simulink model "tractor_mu1109"  (R2022b)
settings: Solver=FixedStepDiscrete  StartTime=0.0  StopTime=20  FixedStep=0.001  RelTol=1e-3
model workspace (MAT data in the model file):
  P : object (value not decoded)
  w_2 : Simulink.Parameter (value not decoded)
undefined symbols (not defined in the file): A, a, B, b, C, D, DiscIntNeverNeededParam, Iz, K, k1, K1, k2, K2, L1, L2, m, magnitude, Phi, Sample_time, Steer_Ratio
libraries: simulink x26, slpidlib x13, Solver_SF x1, dsparch4 x1
(part 5 of 7)

== matlab function tractor_mu1109/Dugoff轮胎模型/pac2002/fr_dugoff ==
  data: Fz input; Fx0 output; u input; lamda input; alpha input; Fy0 output; Fx output; Fy output
function [Fx0,Fy0,Fx,Fy] = tire(Fz,u,lamda,alpha)
cx = -20;
cy = -20;
L = (1-lamda)/(2*sqrt((cx^2)*(lamda^2)+(cy^2)*((tan(alpha))^2)));
if L<1
    fL = L*(2-L);
else
    fL = 1;
end
Fx0 = Fz*cx*lamda*fL/(1-lamda);
Fy0 = Fz*cy*tan(alpha)*fL/(1-lamda);
Fx = u*Fx0;
Fy = u*Fy0;

== matlab function tractor_mu1109/软土分配策略/MATLAB Function1 ==
  data: measured_kappa input; torque_l1_n_m output; baseline_torques_n_m input; wheel_torque_limits_n_m input; torque_r1_n_m output; torque_l2_n_m output; torque_r2_n_m output
function [torque_l1_n_m, torque_r1_n_m, torque_l2_n_m, torque_r2_n_m] = shiche_soft_soil_adaptive_allocation(measured_kappa, baseline_torques_n_m, wheel_torque_limits_n_m)
%SHICHE_SOFT_SOIL_ADAPTIVE_ALLOCATION Direct-slip zero-sum torque allocator.
%
% MATLAB Function block version for real-vehicle VCU code generation. All
% calculations and outputs use single precision.
%
% Wheel vector order:
%   [L1, R1, L2, R2] = [left-front, right-front, left-rear, right-rear]
%
% Inputs:
%   measured_kappa       Directly measured four-wheel longitudinal slip ratios.
%   baseline_torques_n_m Upstream baseline wheel torques in N*m.
%   wheel_torque_limits_n_m Nonnegative maximum wheel torques in N*m.
%
% Outputs:
%   torque_l1_n_m Redistributed left-front wheel torque in N*m.
%   torque_r1_n_m Redistributed right-front wheel torque in N*m.
%   torque_l2_n_m Redistributed left-rear wheel torque in N*m.
%   torque_r2_n_m Redistributed right-rear wheel torque in N*m.
%
% Allocation principle:
%   1. Compare each wheel slip with the four-wheel mean slip.
%   2. Remove torque from wheels with above-average slip and add torque to
%      wheels with below-average slip.
%   3. Limit each wheel's redistribution correction to +/-2600 N*m.
%   4. Force the four correction values to sum to zero, so the final total
%      torque equals the baseline total torque.
%   5. Uniformly reduce the zero-sum correction when needed so every final
%      wheel torque remains between zero and its input wheel torque limit.
%
% This function intentionally contains no slip estimation, adaptive target,
% CBF, QP, or persistent cross-step state.
%
% The baseline allocation is expected to satisfy the input wheel limits. If
% the baseline itself is outside those limits, preserving its total torque and
% satisfying every wheel limit may be impossible. In that case this function
% returns the baseline unchanged and performs no slip redistribution.

slips = reshape(single(measured_kappa), 1, 4);
base_torques = reshape(single(baseline_torques_n_m), 1, 4);
wheel_limits = reshape(single(wheel_torque_limits_n_m), 1, 4);

feedback_gain_n_m = single(20500.0);
correction_limit_n_m = single(2600.0);
corrections = zeros(1, 4, 'single');

% Invalid direct-slip or limit input must not corrupt the baseline allocation.
inputs_valid = true;
baseline_within_limits = true;
for index = 1:4
    if ~isfinite(slips(index)) || ~isfinite(wheel_limits(index)) ...
            || wheel_limits(index) < single(0.0)
        inputs_valid = false;
    end
    if ~isfinite(base_torques(index)) || base_torques(index) < single(0.0) ...
            || base_torques(index) > wheel_limits(index)
        baseline_within_limits = false;
    end
end

if inputs_valid && baseline_within_limits
    mean_slip = sum(slips) / single(4.0);

    % Initial proportional redistribution. Positive slip deviation removes
    % torque; negative slip deviation adds torque.
    for index = 1:4
        slip_deviation = slips(index) - mean_slip;
        corrections(index) = clamp_local( ...
            -feedback_gain_n_m * slip_deviation, ...
            -correction_limit_n_m, ...
            correction_limit_n_m);
    end

    % Independent saturation can make the corrections non-zero-sum. Center
    % them again so torque removed from high-slip wheels is exactly reassigned
    % to lower-slip wheels.
    mean_correction = sum(corrections) / single(4.0);
    for index = 1:4
        corrections(index) = corrections(index) - mean_correction;
    end

    % Re-centering can increase one correction beyond the requested limit.
    % Uniform scaling preserves the zero-sum property and relative allocation.
    maximum_abs_correction = single(0.0);
    for index = 1:4
        maximum_abs_correction = max( ...
            maximum_abs_correction, abs(corrections(index)));
    end
    if maximum_abs_correction > correction_limit_n_m
        scale = correction_limit_n_m / maximum_abs_correction;
        corrections = corrections * scale;
    end

    % Apply one common scale to all corrections so the zero-sum transfer and
    % total baseline torque are preserved while respecting every wheel limit.
    bound_scale = single(1.0);
    for index = 1:4
        if corrections(index) > single(0.0)
            available_increase = wheel_limits(index) - base_torques(index);
            bound_scale = min(bound_scale, available_increase / corrections(index));
        elseif corrections(index) < single(0.0)
            available_decrease = base_torques(index);
            bound_scale = min(bound_scale, available_decrease / -corrections(index));
        end
    end
    bound_scale = clamp_local(bound_scale, single(0.0), single(1.0));
    corrections = corrections * bound_scale;
end

selected_torques = base_torques + corrections;

% Compensate the small single-precision summation residual on a wheel that has
% room in the required direction, without violating an input torque limit.
total_residual = sum(base_torques) - sum(selected_torques);
if inputs_valid && baseline_within_limits && total_residual ~= single(0.0)
    for index = 1:4
        corrected = selected_torques(index) + total_residual;
        if corrected >= single(0.0) && corrected <= wheel_limits(index)
            selected_torques(index) = corrected;
            break;
        end
    end
end

torque_l1_n_m = single(selected_torques(1));
torque_r1_n_m = single(selected_torques(2));
torque_l2_n_m = single(selected_torques(3));
torque_r2_n_m = single(selected_torques(4));
end

function value = clamp_local(value_in, lower, upper)
value = min(max(single(value_in), single(lower)), single(upper));
end

== matlab function tractor_mu1109/软土扭矩分配/状态接口与轮端动力学 ==
  data: wheel_speeds_rpm input; kappa output; front_steer_angles_deg input; longitudinal_speed_mps input; slip_ratios input; slip_ratio_dots input; slip_valid input; baseline_torques_n_m input; wheel_torque_limits_n_m input; dot_kappa output; kappa_valid output; wheel_omegas_radps output; rolling_speeds_mps output; surface_speeds_mps output; front_steers_rad output; base_torques_n_m output; wheel_limits_n_m output; input_gains output
function [kappa, dot_kappa, kappa_valid, wheel_omegas_radps, rolling_speeds_mps, surface_speeds_mps, front_steers_rad, base_torques_n_m, wheel_limits_n_m, input_gains] = MF_StateKinematicsAndGain(wheel_speeds_rpm, front_steer_angles_deg, longitudinal_speed_mps, slip_ratios, slip_ratio_dots, slip_valid, baseline_torques_n_m, wheel_torque_limits_n_m)

% 状态接口与轮端运动学模块
%
% 本模块不再内部估计滑移率。
% 滑移率、滑移率变化率以及滑移率有效标志均由外部状态估计模块输入。
%
% 四轮顺序：
% 1：左前轮
% 2：右前轮
% 3：左后轮
% 4：右后轮

%% 输入整理

wheel_speeds = row4_local(wheel_speeds_rpm);
kappa_input = row4_local(slip_ratios);
dot_kappa_input = row4_local(slip_ratio_dots);
valid_input = row4_local(slip_valid);
base_input = row4_local(baseline_torques_n_m);
limit_input = row4_local(wheel_torque_limits_n_m);

vx = double(longitudinal_speed_mps);

%% 前轮转角整理

front_steers_rad = front_steer_pair_rad_local(front_steer_angles_deg);

%% 基本车辆参数

rpm_to_rad = 2.0 * pi / 60.0;

radii = [0.834, 0.834, 0.94, 0.94];
inertias = [110.64, 110.64, 356.42, 356.42]; % 转动惯量

%% 滑移率外部输入整理

kappa = zeros(1, 4);
dot_kappa = zeros(1, 4);
kappa_valid = zeros(1, 4);

for index = 1:4

    % 外部滑移率直接使用，但做基本数值限幅，防止异常值进入控制器。
    kappa(index) = clamp_local(kappa_input(index), -1.0, 1.0);

    % 外部滑移率变化率直接使用。
    dot_kappa(index) = dot_kappa_input(index);

    % 有效性由外部 slip_valid 给出，同时内部补充有限性检查。
    if valid_input(index) > 0.5 && isfinite(kappa(index)) && isfinite(dot_kappa(index))
        kappa_valid(index) = 1.0;
    else
        kappa_valid(index) = 0.0;
        dot_kappa(index) = 0.0;
    end
end

%% 轮端运动学计算

% 轮速由 rpm 转为 rad/s。
wheel_omegas_radps = abs(wheel_speeds) * rpm_to_rad;

% 车轮圆周速度 v = r * omega。
surface_speeds_mps = radii .* wheel_omegas_radps;

% 车速取绝对值，避免倒车时符号影响滑移率输入增益计算。
speed_abs = abs(vx);

% 前轮转角。
delta_l = front_steers_rad(1);
delta_r = front_steers_rad(2);

% 各轮沿滚动方向的车辆速度。
% 前轮考虑转角投影，后轮无转角。
rolling_speeds_mps = zeros(1, 4);
rolling_speeds_mps(1) = abs(speed_abs * cos(delta_l));
rolling_speeds_mps(2) = abs(speed_abs * cos(delta_r));
rolling_speeds_mps(3) = speed_abs;
rolling_speeds_mps(4) = speed_abs;

%% 基线扭矩与轮端限幅整理

wheel_limits_n_m = zeros(1, 4);
base_torques_n_m = zeros(1, 4);

for index = 1:4

    % 轮端最大扭矩不能为负。
    wheel_limits_n_m(index) = max(0.0, limit_input(index));

    % 基线扭矩限制在物理可行范围内。
    base_torques_n_m(index) = clamp_local(base_input(index), 0.0, wheel_limits_n_m(index));
end

%% 滑移率动力学输入增益计算

% 滑移率动力学近似写为：
% dot(kappa_i) = g_i * T_i + d_i
%
% 其中：
% g_i = v_i / (J_i * r_i * omega_i^2)

input_gains = NaN(1, 4);

for index = 1:4

    if kappa_valid(index) > 0.5 && wheel_omegas_radps(index) > 0.0 && isfinite(rolling_speeds_mps(index))

        gain = rolling_speeds_mps(index) / ...
            (inertias(index) * radii(index) * wheel_omegas_radps(index) * wheel_omegas_radps(index));

        if gain >= 1.0e-8 && isfinite(gain)
            input_gains(index) = gain;
        end
    end
end

end


function output = row4_local(values)

% 将输入信号整理为 1×4 行向量。

input_values = double(values);
output = zeros(1, 4);

for index = 1:4
    output(index) = input_values(index);
end

end


function front_steers_rad = front_steer_pair_rad_local(front_steer_angles_deg)

% 将前轮转角输入整理为左右前轮两个转角，单位 rad。
% 如果输入为两个元素，则分别为左前轮和右前轮转角；
% 如果输入为一个元素，则左右前轮使用同一等效转角。

steer_input = double(front_steer_angles_deg);
front_steers_rad = zeros(1, 2);

if numel(steer_input) >= 2
    front_steers_rad(1) = steer_input(1) * pi / 180.0;
    front_steers_rad(2) = steer_input(2) * pi / 180.0;
else
    front_steers_rad(1) = steer_input(1) * pi / 180.0;
    front_steers_rad(2) = steer_input(1) * pi / 180.0;
end

end


function value = clamp_local(value_in, lower, upper)

% 数值限幅函数。

value = min(max(double(value_in), double(lower)), double(upper));

end

== matlab function tractor_mu1109/四轮转矩分配/基线垂直载荷分配 ==
  data: Mz input; Tfl output; Tfr output; Trl output; Trr output; T0 input; derta input; k input; mode input
function [Tfl,Tfr,Trl,Trr] = fcn(Mz,T0,derta,k,mode)
rf = single(0.834);
rr = single(0.94);
df = single(2.39);
dr = single(2.33);
a = single(2.043);

Trr = single(0);
Trl = single(0);
Tfl = single(0);
Tfr = single(0);


% 强制将输入 Mz 类型设为 single，避免隐式转换
Mz = single(Mz);
T0 = single(T0);
derta = single(derta);
mode = single(mode);

% if mode == 5 || mode == 6
%     k = single(3/7); 
% elseif mode == 1 || mode == 3 
%     k = min(k,1);
%     k = max(k,0.3);
% end

A = T0 / (k + single(1));
B = (Mz - a*sin(derta)*k*A/rf) / (df*cos(derta)*k*rr + dr*rf) * (2*rf*rr);
Trr = (A + B) / single(2);
Trl = (A - B) / single(2);
Tfl = k * Trl;
Tfr = k * Trr;

== matlab function tractor_mu1109/牵引效率计算/右后轮 ==
  data: Tw input; Fx_est output; omega_meas input; Fz input; Fx_raw output; Fx_limited output; omega_hat_out output; e_omega output; wv output
function [Fx_est, Fx_raw, Fx_limited, omega_hat_out, e_omega, wv] = ...
    RearWheelFxObserver(Tw, omega_meas, Fz)

%#codegen
% 单轮纵向驱动力观测器
% 输入仅保留时变信号：
%   Tw         : 轮端驱动力矩 [N*m]
%   omega_meas : 实测车轮角速度 [rad/s]
%   Fz         : 单轮垂直载荷 [N]
%
% 输出：
%   Fx_est        : 最终纵向驱动力估计 [N]
%   Fx_raw        : 原始观测力估计 [N]
%   Fx_limited    : 限幅后力估计 [N]
%   omega_hat_out : 观测器内部估计轮速 [rad/s]
%   e_omega       : 轮速误差 [rad/s]
%   wv            : 低速平滑权重 [-]

% =========================================================
% 1. 固定参数区：根据具体车轮统一在这里调整
% =========================================================

Re = 0.94;              % 有效滚动半径 [m]
Jw = 356.42;            % 车轮等效转动惯量 [kg*m^2]
Ts = 0.001;             % 采样周期 [s]

mu = 0.7;               % 等效附着系数 [-]

l_omega = 50.0;         % 轮速误差反馈增益
fF = 3.0;               % 轮胎力观测带宽 [Hz]
gamma_F = Jw / Re * (2*pi*fF)^2;

enable_smc = 0;         % 是否启用滑模鲁棒项：1启用，0关闭
phi = 1.5;              % 滑模边界层厚度 [rad/s]
Func_ratio = 0.10;      % 未建模力比例，建议0.05~0.20
ks = Re / Jw * Func_ratio * mu * max(Fz, 0.0);

enable_lpf = 0;         % 是否启用输出低通：1启用，0关闭
tau_F = 0.08;           % 输出低通时间常数 [s]

v0 = 0.10;              % 低速权重起点 [m/s]
v1 = 0.80;              % 低速权重终点 [m/s]

eps_neg = 0.0;          % 允许负驱动力比例；严格驱动力估计取0
T_offset = 0.0;         % 轮端扭矩零偏 [N*m]
T_dead = 10.0;          % 扭矩死区 [N*m]

allow_brake_force = 0;  % 0：只估计驱动力；1：允许估计制动力

% =========================================================
% 2. 持久状态变量
% =========================================================

persistent omega_hat
persistent Fx_hat
persistent Fx_filt
persistent initialized

if isempty(initialized)
    omega_hat = 0.0;
    Fx_hat = 0.0;
    Fx_filt = 0.0;
    initialized = false;
end

if ~initialized
    omega_hat = omega_meas;
    Fx_hat = 0.0;
    Fx_filt = 0.0;
    initialized = true;
end

% =========================================================
% 3. 参数保护
% =========================================================

Jw_safe = max(Jw, 1e-6);
Re_safe = max(Re, 1e-6);
Ts_safe = max(Ts, 1e-6);
phi_safe = max(phi, 1e-6);
tau_safe = max(tau_F, Ts_safe);

Fz_safe = max(Fz, 0.0);
mu_safe = max(mu, 0.0);

if v1 <= v0
    v1_safe = v0 + 1e-3;
else
    v1_safe = v1;
end

% =========================================================
% 4. 扭矩零偏与死区处理
% =========================================================

Tw_corr = Tw - T_offset;

if abs(Tw_corr) < T_dead
    Tw_eff = 0.0;
else
    if Tw_corr > 0.0
        Tw_eff = Tw_corr - T_dead;
    else
        Tw_eff = Tw_corr + T_dead;
    end
end

if allow_brake_force < 0.5
    if Tw_eff < 0.0
        Tw_eff = 0.0;
    end
end

% =========================================================
% 5. 轮速误差
% =========================================================

e_omega = omega_meas - omega_hat;

% =========================================================
% 6. 滑模鲁棒项
% =========================================================

s = e_omega / phi_safe;

if s > 1.0
    sat_s = 1.0;
elseif s < -1.0
    sat_s = -1.0;
else
    sat_s = s;
end

if enable_smc > 0.5
    smc_term = ks * sat_s;
else
    smc_term = 0.0;
end

% =========================================================
% 7. 观测器状态更新
% =========================================================
%
% omega_hat_dot = Tw/Jw - Re/Jw*Fx_hat + l_omega*e_omega + ks*sat(e/phi)
% Fx_hat_dot    = -gamma_F*e_omega

omega_hat_dot = ...
    Tw_eff / Jw_safe ...
    - Re_safe / Jw_safe * Fx_hat ...
    + l_omega * e_omega ...
    + smc_term;

Fx_hat_dot = -gamma_F * e_omega;

omega_hat = omega_hat + Ts_safe * omega_hat_dot;
Fx_hat = Fx_hat + Ts_safe * Fx_hat_dot;

% =========================================================
% 8. 物理限幅与抗积分发散
% =========================================================

Fx_max = mu_safe * Fz_safe;

if allow_brake_force > 0.5
    Fx_min = -mu_safe * Fz_safe;
else
    Fx_min = -eps_neg * Fz_safe;
end

if Fx_hat > Fx_max
    Fx_hat = Fx_max;
elseif Fx_hat < Fx_min
    Fx_hat = Fx_min;
end

Fx_raw = Fx_hat;

if Fx_raw > Fx_max
    Fx_limited = Fx_max;
elseif Fx_raw < Fx_min
    Fx_limited = Fx_min;
else
    Fx_limited = Fx_raw;
end

% =========================================================
% 9. 低速平滑权重
% =========================================================

vw = abs(Re_safe * omega_meas);

wv = (vw - v0) / (v1_safe - v0);

if wv > 1.0
    wv = 1.0;
elseif wv < 0.0
    wv = 0.0;
end

wv = wv * wv * (3.0 - 2.0 * wv);

Fx_weighted = wv * Fx_limited;

% =========================================================
% 10. 输出低通滤波
% =========================================================

if enable_lpf > 0.5
    alpha = exp(-Ts_safe / tau_safe);
    Fx_filt = alpha * Fx_filt + (1.0 - alpha) * Fx_weighted;
    Fx_est = Fx_filt;
else
    Fx_filt = Fx_weighted;
    Fx_est = Fx_weighted;
end

omega_hat_out = omega_hat;

end

== matlab function tractor_mu1109/Dugoff轮胎模型/pac2002/rl_dugoff ==
  data: Fz input; Fx0 output; u input; lamda input; alpha input; Fy0 output; Fx output; Fy output
function [Fx0,Fy0,Fx,Fy] = tire(Fz,u,lamda,alpha)
cx = -20;
cy = -20;
L = (1-lamda)/(2*sqrt(cx^2*lamda^2+cy^2*(tan(alpha))^2));
if L<1
    fL = L*(2-L);
else
    fL = 1;
end
Fx0 = Fz*cx*lamda*fL/(1-lamda);
Fy0 = Fz*cy*tan(alpha)*fL/(1-lamda);
Fx = u*Fx0;
Fy = u*Fy0;

== matlab function tractor_mu1109/Dugoff轮胎模型/pac2002/rr_dugoff ==
  data: Fz input; Fx0 output; u input; lamda input; alpha input; Fy0 output; Fx output; Fy output
function [Fx0,Fy0,Fx,Fy] = tire(Fz,u,lamda,alpha)
cx = -20;
cy = -20;
L = (1-lamda)/(2*sqrt((cx^2)*(lamda^2)+(cy^2)*((tan(alpha))^2)));
if L<1
    fL = L*(2-L);
else
    fL = 1;
end
Fx0 = Fz*cx*lamda*fL/(1-lamda);
Fy0 = Fz*cy*tan(alpha)*fL/(1-lamda);
Fx = u*Fx0;
Fy = u*Fy0;

== matlab function tractor_mu1109/质心侧偏角估计/define_Kalman ==
  data: u input; A output; B output; C output; D output; a11 output; a12 output; a21 output single; a22 output; c11 output; c12 output
function [A, B, C, D,a11,a12,a21,a22,c11,c12] = fcn(u)
m = 18530;%质量
Iz = 67536;%绕Z轴的转动惯量
a = 2.043;%前轴距
b=1.362;%后轴距
% k1 = -1360400;%前侧偏刚度
% k2 = -1611200;%后侧偏刚度
k1 = -304828*2;%前侧偏刚度
k2 = -417040*2;%后侧偏刚度
t = 0.001;%仿真步长
Sample_time = 0.001;


a11 = (k1+k2)*t/(m*u)+1;
a12 = ((a*k1-b*k2)/(m*u^2)-1)*t;
a21 = single((a*k1-b*k2)*t/Iz);
a22 = (a^2*k1+b^2*k2)*t/(Iz*u)+1;
b11  =-k1*t/(m*u);
b21 = -a*k1*t/Iz;
c11 = (k1+k2)/m;
c12 = (a*k1-b*k2)/(m*u);
c21 = 0;
c22 = 1;
d11 = -k1/m;
d21 = 0;

%% A B C D 为kalman滤波器中各个矩阵

A = [a11 a12;a21 a22];
B = [b11;b21];
C = [c11 c12;c21 c22];
D = [d11;d21];

== matlab function tractor_mu1109/驱动防滑模块/MATLAB Function ==
  data: sp1 input; vfl output; sp2 input; vfr output
function [vfl,vfr] = fcn(sp1,sp2)
r1 = 0.834;

if sp1>=0
    vfl = max(0.001,sp1*2*pi*r1/60); %m/s
else
    vfl = min(-0.001,sp1*2*pi*r1/60); %m/s
end

if sp2 >= 0
    vfr = max(0.001,sp2*2*pi*r1/60);
else
    vfr = min(0.001,sp2*2*pi*r1/60);
end

== matlab function tractor_mu1109/驱动防滑模块/MATLAB Function1 ==
  data: sp3 input; vrl output; sp4 input; vrr output
function [vrl,vrr] = fcn(sp3,sp4)
r2 = 0.94;

if sp3 >= 0
    vrl = max(0.001,sp3*2*pi*r2/60);
else
    vrl = min(0.001,sp3*2*pi*r2/60);
end

if sp4 >=0
    vrr = max(0.001,sp4*2*pi*r2/60);
else
    vrr = min(0.001,sp4*2*pi*r2/60);
end

== stateflow chart tractor_mu1109/驱动防滑模块/转矩协调控制 ==
  state coordinate
    (default) -> (junction 7)
    (junction 7) -> (junction 9) [order 1] : [dT1 ~= 0]
    (junction 9) -> (junction 11) [order 1] : [dT2 ~= 0]
    (junction 11) -> (junction 14) [order 1] : [abs(dT1)>=abs(dT2)]{dTfr=dT1;dTfl=dT1;}
    (junction 14) -> (junction 16)
    (junction 7) -> (junction 21) [order 2] : {dTfr=dT2;
        | dTfl=dT2}
    (junction 9) -> (junction 19) [order 2] : {dTfr=dT1;
        | dTfl=dT1;}
    (junction 11) -> (junction 16) [order 2] : {dTfr=dT2;dTfl=dT2;}
    (junction 19) -> (junction 21)
    (junction 16) -> (junction 19)
    (junction 21) -> (junction 111)
    (junction 111) -> (junction 106) [order 2] : {dTrr=dT4;
        | dTrl=dT4}
    (junction 111) -> (junction 118) [order 1] : [dT3 ~= 0]
    (junction 118) -> (junction 107) [order 1] : [dT4 ~= 0]
    (junction 107) -> (junction 110) [order 1] : [abs(dT3)>=abs(dT4)]{dTrr=dT3;dTrl=dT3;}
    (junction 110) -> (junction 114)
    (junction 115) -> (junction 106)
    (junction 118) -> (junction 115) [order 2] : {dTrr=dT3;
        | dTrl=dT3;}
    (junction 107) -> (junction 114) [order 2] : {dTrr=dT4;dTrl=dT4;}
    (junction 114) -> (junction 115)
  state no_coordinate
    du:
    dTfl=dT1;
    dTfr=dT2;
    dTrl=dT3;
    dTrr=dT4;
  (default) -> (junction 123)
  (junction 123) -> (junction 126) [order 2]
  (junction 123) -> no_coordinate [order 1] : [v<10]
  (junction 126) -> coordinate
  no_coordinate -> coordinate : [v>=10]
  coordinate -> no_coordinate [order 1] : [v<10]
  coordinate -> coordinate [order 2] : [v>=10]
  data: v input; dT1 input; dT2 input; dT3 input; dT4 input; dTfl output; dTfr output; dTrl output; dTrr output

== matlab function tractor_mu1109/四轮转矩分配/MATLAB Function1 ==
  data: X_current input; U_optimal output; Fx input; Mz input; Fz_all input; mu input; last_U_in input
function U_optimal = mpc_torque_allocation_fcn(X_current, Fx, Mz, Fz_all, mu, last_U_in)
% 基于MPC的四轮驱动车辆扭矩分配。
% 本函数在每个计算步中构建并求解一个二次规划(QP)问题。

%#codegen

% -------------------------------------------------------------------------
% 1. 定义持久化变量和参数
% -------------------------------------------------------------------------
% persistent 关键字定义的变量只在第一次调用函数时初始化，之后会保持它们的值。
persistent vehicle_params mpc_params last_U

if isempty(vehicle_params)
    % --- 车辆参数 ---
    % !! 请根据您的拖拉机模型修改以下参数 !!
    vehicle_params.m = 18530;   % 质量 (kg)
    vehicle_params.Iz = 67536;  % 绕Z轴的转动惯量 (kg*m^2)
    vehicle_params.lf = 2.043;   % 质心到前轴的距离 (m)
    vehicle_params.lr = 1.362;   % 质心到后轴的距离 (m)
    vehicle_params.wf = 2.39;    % 前轮距 (m)
    vehicle_params.wr = 2.33;    % 后轮距 (m)

    % --- MPC 参数 ---
    mpc_params.Ts = 0.001;      % 采样时间 (s)，必须与Simulink的采样时间一致
    mpc_params.Np = 20;        % 预测时域 (Prediction Horizon)
    mpc_params.Nc = 10;         % 控制时域 (Control Horizon)
    
    % --- MPC 权重 ---
    % 对控制输入变化率 (delta U) 的惩罚矩阵R的对角线元素
    mpc_params.R_diag = ones(8, 1) * 0.01; 
    mpc_params.w_ax = 1.0;      % 纵向加速度权重
    mpc_params.w_ay = 1;      % 横向加速度权重
    
    % --- 轮胎附着多边形 ---
    % 使用一个八边形来线性化近似摩擦圆约束
    num_sides = 8;
    angles = (0:num_sides-1)' * (2*pi/num_sides);
    mpc_params.friction_polygon = [cos(angles), sin(angles)]; % [cos, sin] 列
    
    % 初始化上一次的控制输入
    last_U = zeros(8, 1);
end

% 从输入端口更新last_U，以保证时间步之间的一致性
if any(size(last_U_in) ~= size(last_U))
   last_U = zeros(8,1); % 如果是第一次运行或尺寸不匹配，则进行初始化
else
   last_U = last_U_in;
end


% -------------------------------------------------------------------------
% 2. 获取参数
% -------------------------------------------------------------------------
% 车辆参数
m = vehicle_params.m;
Iz = vehicle_params.Iz;
lf = vehicle_params.lf;
lr = vehicle_params.lr;
wf = vehicle_params.wf;
wr = vehicle_params.wr;
bf = wf / 2; % 半轮距
br = wr / 2;

% MPC参数
Ts = mpc_params.Ts;
Np = mpc_params.Np;
Nc = mpc_params.Nc;
R = diag(mpc_params.R_diag);

% 解析输入信号
u_k = X_current(1); % 当前的纵向车速 (m/s)
v_k = X_current(2); % 当前的横向车速 (m/s)
r_k = X_current(3); % 当前横摆角速度 (rad/s)

% -------------------------------------------------------------------------
% 3. 定义状态空间矩阵 
% -------------------------------------------------------------------------
% 连续时间的状态矩阵 A_c，它依赖于当前车速 u_k
A_c = [0, 0, 0;
       0, 0, u_k;
       0, 0, 0];

% 连续时间的输入矩阵 B_c  横摆方向逆时针为正;横向向左为正
B_c = [1/m,   0,   1/m,   0,   1/m,   0,   1/m,   0;
       0,   1/m,   0,   1/m,   0,   1/m,   0,   1/m;
       -bf/Iz, lf/Iz, bf/Iz, lf/Iz, -br/Iz, -lr/Iz, br/Iz, -lr/Iz];

% 使用前向欧拉法进行离散化
Ad = eye(3) + A_c * Ts;
Bd = B_c * Ts;

% -------------------------------------------------------------------------
% 4. 构建二次规划(QP)问题 
%    目标: min 0.5 * dU' * H * dU + f' * dU
% -------------------------------------------------------------------------
% 新代价函数: J = sum( (ax^2+ay^2) + dU'*R*dU )

% ---- 4.1 定义权重和矩阵 ----
% 从参数区获取加速度权重
w_ax = mpc_params.w_ax;
w_ay = mpc_params.w_ay;
Q_accel = diag([w_ax^2, w_ay^2]); % 单步的加速度权重矩阵

% 构建整个控制时域的权重矩阵
Q_bar = kron(eye(Nc), Q_accel);  % 加速度项的权重矩阵
R_bar = kron(eye(Nc), R);      % 控制增量项的权重矩阵

% ---- 4.2 将加速度表示为dU的函数 ----
% 定义一个矩阵，从控制向量U中提取与加速度相关的力
C_u = [1/m, 0, 1/m, 0, 1/m, 0, 1/m, 0;
       0, 1/m, 0, 1/m, 0, 1/m, 0, 1/m];
C_u_bar = kron(eye(Nc), C_u);

% 计算由当前状态(u_k, v_k, r_k)引起的加速度偏移量
% (在线性化过程中被视为常数)
d_accel_k = [-v_k * r_k; 2 * u_k * r_k];
d_accel_bar = repmat(d_accel_k, Nc, 1);

% ---- 4.3 构建QP矩阵 H 和 f ----
% 回忆: U_vec = M_sum * dU_vec + U_last_vec
% 预测的加速度 Accel_vec = C_u_bar * U_vec + d_accel_bar
%                        = C_u_bar * (M_sum * dU_vec + U_last_vec) + d_accel_bar
%                        = (C_u_bar * M_sum) * dU_vec + (C_u_bar * U_last_vec + d_accel_bar)
%
% 令 S = C_u_bar * M_sum
% 令 E = C_u_bar * U_last_vec + d_accel_bar
% 则 Accel_vec = S * dU_vec + E
%
% 加速度部分的代价 J_accel = (S*dU+E)' * Q_bar * (S*dU+E)
% 展开后与QP标准型对比，可以推导出H和f的构成

% 预先计算一个将 dU_vec 映射到 U_vec 的矩阵
% U_vec = M_sum * dU_vec + U_last_vec
M_sum = kron(tril(ones(Nc, Nc)), eye(8));
U_last_vec = repmat(last_U, Nc, 1);

S = C_u_bar * M_sum;
E = C_u_bar * U_last_vec + d_accel_bar;

% 构建 H 矩阵
H = 2 * (S' * Q_bar * S + R_bar);

% 构建 f 向量
f = 2 * (S' * Q_bar * E);

% ---- 4.2 构建约束矩阵 ----
% 优化变量是dU。所有约束都必须是关于dU的线性形式: A*dU <= b 或 Aeq*dU = beq
% 未来的控制量 U_k+i 与 增量 dU 的关系: U_k+i = U_{k-1} + dU_k + ... + dU_k+i



% --- 4.2.1 等式约束: Aeq * dU_vec = beq ---
% 在所有 Nc 控制步内，都满足 Fx_total = Fx_ref 和 Mz_total = Mz_ref
C_fx = [1, 0, 1, 0, 1, 0, 1, 0];
C_mz = [-bf, lf, bf, lf, -br, -lr, br, -lr]; % 注意: 此处未除以Iz，因为约束是针对力矩本身

Aeq_block = [C_fx; C_mz]; % (维度: 2 x 8)
Aeq = kron(eye(Nc), Aeq_block); % (维度: 2*Nc x 8*Nc)
Aeq = Aeq * M_sum;

% 构建等式约束右侧的beq向量
beq_fx = ones(Nc, 1) * Fx;
beq_mz = ones(Nc, 1) * Mz;
beq_block = [beq_fx'; beq_mz']; % (维度: 2 x Nc)
beq = beq_block(:); % (维度: 2*Nc x 1)
% 别忘了减去上个时刻控制量的影响
beq = beq - kron(eye(Nc), Aeq_block) * U_last_vec;

% --- 4.2.2 不等式约束: Aineq * dU_vec <= bineq ---
% 对所有4个轮胎、在所有Nc控制步内的轮胎附着多边形约束
% poly_sides = mpc_params.friction_polygon;
% num_sides = size(poly_sides, 1);
% num_tires = 4;
% 
% Aineq_block = zeros(num_sides * num_tires, 8);
% for i = 1:num_tires % 遍历: 左前, 右前, 左后, 右后
%     % 找到这个轮胎对应的Fx和Fy列的索引
%     idx_fx = 2*i - 1;
%     idx_fy = 2*i;
%     
%     % 获取这个轮胎对应约束的行索引范围
%     row_start = (i-1)*num_sides + 1;
%     row_end = i*num_sides;
%     
%     % 填充多边形约束系数
%     Aineq_block(row_start:row_end, idx_fx) = poly_sides(:, 1); % cos(theta)
%     Aineq_block(row_start:row_end, idx_fy) = poly_sides(:, 2); % sin(theta)
% end
% 
% Aineq = kron(eye(Nc), Aineq_block); % (维度: num_sides*num_tires*Nc x 8*Nc)
% Aineq = Aineq * M_sum;
% 
% % 构建不等式约束右侧的bineq向量
% mu_vec = ones(4,1) * mu; % 暂时假设所有轮胎的附着系数 mu 相同
% Fz_mu_vec = Fz_all .* mu_vec; % 计算每个轮胎的最大附着力
% bineq_block = repelem(Fz_mu_vec, num_sides, 1); % repelem for R2017a+, for older use kron
% bineq = repmat(bineq_block, Nc, 1);
% % 同样，减去上个时刻控制量的影响
% bineq = bineq - kron(eye(Nc), Aineq_block) * U_last_vec;

% -------------------------------------------------------------------------
% 5. 求解QP问题
% -------------------------------------------------------------------------
% 设置 quadprog 求解器选项
U_optimal = zeros(8,1);
options = optimoptions('quadprog', 'Display', 'none', 'Algorithm', 'active-set');

% 为求解器创建一个全零的初始猜测点 x0
% 它的维度必须与优化变量dU_vec一致 (8*Nc x 1)
x0 = zeros(8 * Nc, 1);

% --- 【新增代码】构建下界(lb)向量以保证驱动轮Fx >= 0 ---
% lb是直接作用于优化变量dU_vec的

% 首先，为单个时间步的dU创建一个下界向量
lb_step = -inf(8, 1);

% 假设所有4个轮子都只作为驱动轮，不能为负
% Fx的索引是 1, 3, 5, 7
drive_idx = [1, 3, 5, 7]; 
% Fx的增量的下界是上一时刻Fx的负值，以保证 Fx_k = Fx_{k-1} + dFx_k >= 0
lb_step(drive_idx) = -last_U(drive_idx);

% 然后，将单步的下界向量复制Nc次，以覆盖整个控制时域
lb = repmat(lb_step, Nc, 1);

% 【修改代码】调用求解器，将lb作为第7个参数传入
% [dU_vec_sol, ~, exitflag] = quadprog(H, f, Aineq, bineq, Aeq, beq, lb, [], x0, options);
[dU_vec_sol, ~, exitflag] = quadprog(H, f, [], [], Aeq, beq, lb, [], x0, options);
% -------------------------------------------------------------------------
% 6. 处理求解结果
% -------------------------------------------------------------------------
if exitflag == 1 % 返回1代表求解成功
    % 提取第一个控制增量 (Receding Horizon Control)
    dU_optimal = dU_vec_sol(1:8);
    % 计算当前时刻的最终控制输入
    U_optimal = last_U + dU_optimal;
else
    % 如果求解失败, 保持上一次的控制输入不变 (作为一种安全备用策略)
    U_optimal = last_U;
end

% 无需在此更新 last_U, 因为它会作为输出连接到Unit Delay模块，
% 并在下个采样时刻通过输入端口 last_U_in 传回。

end

== matlab function tractor_mu1109/牵引效率计算/MATLAB Function ==
  data: Fd input; P_qianyin input; y output; P_qudong input; v input
function y = fcn(Fd,P_qianyin,P_qudong,v)

if Fd > 0 && v > 0.5/3.6
    y = P_qianyin/P_qudong;
else
    y = 0;
end
if P_qudong < 2000
    y = 0;
end

== matlab function tractor_mu1109/四轮转矩分配/MATLAB Function2 ==
  data: F input; Tfl output; derta input; Tfr output; Trl output; Trr output; dwfl input; dwfr input; dwrl input; dwrr input
function [Tfl,Tfr,Trl,Trr] = fcn(F,derta,dwfl,dwfr,dwrl,dwrr)
% 向左为正
rf = 0.834;
rr = 0.94;
If = 110.64; % kg*m^2
Ir = 356.42;

Ffl = F(1)*cos(derta) + F(2)*sin(derta);
Tfl = Ffl*rf + If*dwfl;
Ffr = F(3)*cos(derta) + F(4)*sin(derta);
Tfr = Ffr*rf + If*dwfr;
Frl = F(5);
Trl = Frl*rr + Ir*dwrl;
Frr = F(7);
Trr = Frr*rr + Ir*dwrr;

== matlab function tractor_mu1109/驱动防滑模块/MATLAB Function2 ==
  data: v input; dTfl output; dT1 input; dT2 input; dT3 input; dT4 input; dTfr output; dTrl output; dTrr output
function [dTfl,dTfr,dTrl,dTrr] = fcn(v,dT1,dT2,dT3,dT4)

v = v*3.6;

if v < 1.5
    dTfl = 0;
    dTfr = 0;
    dTrl = 0;
    dTrr = 0;
end

if v < 10
    dTfl = dT1;
    dTfr = dT2;
    dTrl = dT3;
    dTrr = dT4;
else 
    if abs(dT1) > abs(dT2)
        dTfl = dT1;
        dTfr = dT1;
    else
        dTfl = dT2;
        dTfr = dT2;
    end
    if abs(dT3) > abs(dT4)
        dTrl = dT3;
        dTrr = dT3;
    else
        dTrl = dT4;
        dTrr = dT4;
    end
end

== matlab function tractor_mu1109/牵引效率计算/左后轮 ==
  data: Tw input; Fx_est output; omega_meas input; Fz input; Fx_raw output; Fx_limited output; omega_hat_out output; e_omega output; wv output
function [Fx_est, Fx_raw, Fx_limited, omega_hat_out, e_omega, wv] = ...
    RearWheelFxObserver(Tw, omega_meas, Fz)

%#codegen
% 单轮纵向驱动力观测器
% 输入仅保留时变信号：
%   Tw         : 轮端驱动力矩 [N*m]
%   omega_meas : 实测车轮角速度 [rad/s]
%   Fz         : 单轮垂直载荷 [N]
%
% 输出：
%   Fx_est        : 最终纵向驱动力估计 [N]
%   Fx_raw        : 原始观测力估计 [N]
%   Fx_limited    : 限幅后力估计 [N]
%   omega_hat_out : 观测器内部估计轮速 [rad/s]
%   e_omega       : 轮速误差 [rad/s]
%   wv            : 低速平滑权重 [-]

% =========================================================
% 1. 固定参数区：根据具体车轮统一在这里调整
% =========================================================

Re = 0.94;              % 有效滚动半径 [m]
Jw = 356.42;            % 车轮等效转动惯量 [kg*m^2]
Ts = 0.001;             % 采样周期 [s]

mu = 0.7;               % 等效附着系数 [-]

l_omega = 50.0;         % 轮速误差反馈增益
fF = 3.0;               % 轮胎力观测带宽 [Hz]
gamma_F = Jw / Re * (2*pi*fF)^2;

enable_smc = 0;         % 是否启用滑模鲁棒项：1启用，0关闭
phi = 1.5;              % 滑模边界层厚度 [rad/s]
Func_ratio = 0.10;      % 未建模力比例，建议0.05~0.20
ks = Re / Jw * Func_ratio * mu * max(Fz, 0.0);

enable_lpf = 0;         % 是否启用输出低通：1启用，0关闭
tau_F = 0.08;           % 输出低通时间常数 [s]

v0 = 0.10;              % 低速权重起点 [m/s]
v1 = 0.80;              % 低速权重终点 [m/s]

eps_neg = 0.0;          % 允许负驱动力比例；严格驱动力估计取0
T_offset = 0.0;         % 轮端扭矩零偏 [N*m]
T_dead = 10.0;          % 扭矩死区 [N*m]

allow_brake_force = 0;  % 0：只估计驱动力；1：允许估计制动力

% =========================================================
% 2. 持久状态变量
% =========================================================

persistent omega_hat
persistent Fx_hat
persistent Fx_filt
persistent initialized

if isempty(initialized)
    omega_hat = 0.0;
    Fx_hat = 0.0;
    Fx_filt = 0.0;
    initialized = false;
end

if ~initialized
    omega_hat = omega_meas;
    Fx_hat = 0.0;
    Fx_filt = 0.0;
    initialized = true;
end

% =========================================================
% 3. 参数保护
% =========================================================

Jw_safe = max(Jw, 1e-6);
Re_safe = max(Re, 1e-6);
Ts_safe = max(Ts, 1e-6);
phi_safe = max(phi, 1e-6);
tau_safe = max(tau_F, Ts_safe);

Fz_safe = max(Fz, 0.0);
mu_safe = max(mu, 0.0);

if v1 <= v0
    v1_safe = v0 + 1e-3;
else
    v1_safe = v1;
end

% =========================================================
% 4. 扭矩零偏与死区处理
% =========================================================

Tw_corr = Tw - T_offset;

if abs(Tw_corr) < T_dead
    Tw_eff = 0.0;
else
    if Tw_corr > 0.0
        Tw_eff = Tw_corr - T_dead;
    else
        Tw_eff = Tw_corr + T_dead;
    end
end

if allow_brake_force < 0.5
    if Tw_eff < 0.0
        Tw_eff = 0.0;
    end
end

% =========================================================
% 5. 轮速误差
% =========================================================

e_omega = omega_meas - omega_hat;

% =========================================================
% 6. 滑模鲁棒项
% =========================================================

s = e_omega / phi_safe;

if s > 1.0
    sat_s = 1.0;
elseif s < -1.0
    sat_s = -1.0;
else
    sat_s = s;
end

if enable_smc > 0.5
    smc_term = ks * sat_s;
else
    smc_term = 0.0;
end

% =========================================================
% 7. 观测器状态更新
% =========================================================
%
% omega_hat_dot = Tw/Jw - Re/Jw*Fx_hat + l_omega*e_omega + ks*sat(e/phi)
% Fx_hat_dot    = -gamma_F*e_omega

omega_hat_dot = ...
    Tw_eff / Jw_safe ...
    - Re_safe / Jw_safe * Fx_hat ...
    + l_omega * e_omega ...
    + smc_term;

Fx_hat_dot = -gamma_F * e_omega;

omega_hat = omega_hat + Ts_safe * omega_hat_dot;
Fx_hat = Fx_hat + Ts_safe * Fx_hat_dot;

% =========================================================
% 8. 物理限幅与抗积分发散
% =========================================================

Fx_max = mu_safe * Fz_safe;

if allow_brake_force > 0.5
    Fx_min = -mu_safe * Fz_safe;
else
    Fx_min = -eps_neg * Fz_safe;
end

if Fx_hat > Fx_max
    Fx_hat = Fx_max;
elseif Fx_hat < Fx_min
    Fx_hat = Fx_min;
end

Fx_raw = Fx_hat;

if Fx_raw > Fx_max
    Fx_limited = Fx_max;
elseif Fx_raw < Fx_min
    Fx_limited = Fx_min;
else
    Fx_limited = Fx_raw;
end

% =========================================================
% 9. 低速平滑权重
% =========================================================

vw = abs(Re_safe * omega_meas);

wv = (vw - v0) / (v1_safe - v0);

if wv > 1.0
    wv = 1.0;
elseif wv < 0.0
    wv = 0.0;
end

wv = wv * wv * (3.0 - 2.0 * wv);

Fx_weighted = wv * Fx_limited;

% =========================================================
% 10. 输出低通滤波
% =========================================================

if enable_lpf > 0.5
    alpha = exp(-Ts_safe / tau_safe);
    Fx_filt = alpha * Fx_filt + (1.0 - alpha) * Fx_weighted;
    Fx_est = Fx_filt;
else
    Fx_filt = Fx_weighted;
    Fx_est = Fx_weighted;
end

omega_hat_out = omega_hat;

end

== stateflow chart tractor_mu1109/车轮腾空判断/FL ==
  state suspected
    airborne_flag = 0; confidence = 0.5;
  state grounded
    airborne_flag = 0; confidence = 0;
  state airborne
    airborne_flag = 1; confidence = 1;
  grounded -> suspected : [ (lamda > 0) && (Tload_hat < 50) && (domega > 0) && (abs(az)) > 2]
  suspected -> airborne : [after(0.02, sec)]
  (default) -> grounded
  airborne -> grounded : [(lamda < 0.02) && (Tload_hat > 100) && abs(az) < 1 && after(0.05,sec)]
  data: lamda input; Tload_hat input; az input; domega input; airborne_flag output; confidence output

== stateflow chart tractor_mu1109/车轮腾空判断/FR ==
  state suspected
    airborne_flag = 0; confidence = 0.5;
  state grounded
    airborne_flag = 0; confidence = 0;
  state airborne
    airborne_flag = 1; confidence = 1;
  grounded -> suspected : [ (lamda > 0) && (Tload_hat < 50) && (domega > 0) && (abs(az)) > 2]
  suspected -> airborne : [after(0.02, sec)]
  (default) -> grounded
  airborne -> grounded : [(lamda < 0.02) && (Tload_hat > 100) && abs(az) < 1 && after(0.05,sec)]
  data: lamda input; Tload_hat input; az input; domega input; airborne_flag output; confidence output

== stateflow chart tractor_mu1109/车轮腾空判断/RL ==
  state suspected
    airborne_flag = 0; confidence = 0.5;
  state grounded
    airborne_flag = 0; confidence = 0;
  state airborne
    airborne_flag = 1; confidence = 1;
  grounded -> suspected : [ (lamda > 0) && (Tload_hat < 50) && (domega > 0) && (abs(az)) > 2]
  suspected -> airborne : [after(0.02, sec)]
  (default) -> grounded
  airborne -> grounded : [(lamda < 0.02) && (Tload_hat > 100) && abs(az) < 1 && after(0.05,sec)]
  data: lamda input; Tload_hat input; az input; domega input; airborne_flag output; confidence output

== stateflow chart tractor_mu1109/车轮腾空判断/RR ==
  state suspected
    airborne_flag = 0; confidence = 0.5;
  state grounded
    airborne_flag = 0; confidence = 0;
  state airborne
    airborne_flag = 1; confidence = 1;
  grounded -> suspected : [ (lamda > 0) && (Tload_hat < 50) && (domega > 0) && (abs(az)) > 2]
  suspected -> airborne : [after(0.02, sec)]
  (default) -> grounded
  airborne -> grounded : [(lamda < 0.02) && (Tload_hat > 100) && abs(az) < 1 && after(0.05,sec)]
  data: lamda input; Tload_hat input; az input; domega input; airborne_flag output; confidence output

== matlab function tractor_mu1109/牵引效率计算/右前轮 ==
  data: Tw input; Fx_est output; omega_meas input; Fz input; Fx_raw output; Fx_limited output; omega_hat_out output; e_omega output; wv output
function [Fx_est, Fx_raw, Fx_limited, omega_hat_out, e_omega, wv] = ...
    FrontWheelFxObserver(Tw, omega_meas, Fz)

%#codegen
% 单轮纵向驱动力观测器
% 输入仅保留时变信号：
%   Tw         : 轮端驱动力矩 [N*m]
%   omega_meas : 实测车轮角速度 [rad/s]
%   Fz         : 单轮垂直载荷 [N]
%
% 输出：
%   Fx_est        : 最终纵向驱动力估计 [N]
%   Fx_raw        : 原始观测力估计 [N]
%   Fx_limited    : 限幅后力估计 [N]
%   omega_hat_out : 观测器内部估计轮速 [rad/s]
%   e_omega       : 轮速误差 [rad/s]
%   wv            : 低速平滑权重 [-]

% =========================================================
% 1. 固定参数区：根据具体车轮统一在这里调整
% =========================================================

Re = 0.834;              % 有效滚动半径 [m]
Jw = 110.64;            % 车轮等效转动惯量 [kg*m^2]
Ts = 0.001;             % 采样周期 [s]

mu = 0.7;               % 等效附着系数 [-]

l_omega = 50.0;         % 轮速误差反馈增益
fF = 3.0;               % 轮胎力观测带宽 [Hz]
gamma_F = Jw / Re * (2*pi*fF)^2;

enable_smc = 0;         % 是否启用滑模鲁棒项：1启用，0关闭
phi = 1.5;              % 滑模边界层厚度 [rad/s]
Func_ratio = 0.10;      % 未建模力比例，建议0.05~0.20
ks = Re / Jw * Func_ratio * mu * max(Fz, 0.0);

enable_lpf = 0;         % 是否启用输出低通：1启用，0关闭
tau_F = 0.08;           % 输出低通时间常数 [s]

v0 = 0.10;              % 低速权重起点 [m/s]
v1 = 0.80;              % 低速权重终点 [m/s]

eps_neg = 0.0;          % 允许负驱动力比例；严格驱动力估计取0
T_offset = 0.0;         % 轮端扭矩零偏 [N*m]
T_dead = 10.0;          % 扭矩死区 [N*m]

allow_brake_force = 0;  % 0：只估计驱动力；1：允许估计制动力

% =========================================================
% 2. 持久状态变量
% =========================================================

persistent omega_hat
persistent Fx_hat
persistent Fx_filt
persistent initialized

if isempty(initialized)
    omega_hat = 0.0;
    Fx_hat = 0.0;
    Fx_filt = 0.0;
    initialized = false;
end

if ~initialized
    omega_hat = omega_meas;
    Fx_hat = 0.0;
    Fx_filt = 0.0;
    initialized = true;
end

% =========================================================
% 3. 参数保护
% =========================================================

Jw_safe = max(Jw, 1e-6);
Re_safe = max(Re, 1e-6);
Ts_safe = max(Ts, 1e-6);
phi_safe = max(phi, 1e-6);
tau_safe = max(tau_F, Ts_safe);

Fz_safe = max(Fz, 0.0);
mu_safe = max(mu, 0.0);

if v1 <= v0
    v1_safe = v0 + 1e-3;
else
    v1_safe = v1;
end

% =========================================================
% 4. 扭矩零偏与死区处理
% =========================================================

Tw_corr = Tw - T_offset;

if abs(Tw_corr) < T_dead
    Tw_eff = 0.0;
else
    if Tw_corr > 0.0
        Tw_eff = Tw_corr - T_dead;
    else
        Tw_eff = Tw_corr + T_dead;
    end
end

if allow_brake_force < 0.5
    if Tw_eff < 0.0
        Tw_eff = 0.0;
    end
end

% =========================================================
% 5. 轮速误差
% =========================================================

e_omega = omega_meas - omega_hat;

% =========================================================
% 6. 滑模鲁棒项
% =========================================================

s = e_omega / phi_safe;

if s > 1.0
    sat_s = 1.0;
elseif s < -1.0
    sat_s = -1.0;
else
    sat_s = s;
end

if enable_smc > 0.5
    smc_term = ks * sat_s;
else
    smc_term = 0.0;
end

% =========================================================
% 7. 观测器状态更新
% =========================================================
%
% omega_hat_dot = Tw/Jw - Re/Jw*Fx_hat + l_omega*e_omega + ks*sat(e/phi)
% Fx_hat_dot    = -gamma_F*e_omega

omega_hat_dot = ...
    Tw_eff / Jw_safe ...
    - Re_safe / Jw_safe * Fx_hat ...
    + l_omega * e_omega ...
    + smc_term;

Fx_hat_dot = -gamma_F * e_omega;

omega_hat = omega_hat + Ts_safe * omega_hat_dot;
Fx_hat = Fx_hat + Ts_safe * Fx_hat_dot;

% =========================================================
% 8. 物理限幅与抗积分发散
% =========================================================

Fx_max = mu_safe * Fz_safe;

if allow_brake_force > 0.5
    Fx_min = -mu_safe * Fz_safe;
else
    Fx_min = -eps_neg * Fz_safe;
end

if Fx_hat > Fx_max
    Fx_hat = Fx_max;
elseif Fx_hat < Fx_min
    Fx_hat = Fx_min;
end

Fx_raw = Fx_hat;

if Fx_raw > Fx_max
    Fx_limited = Fx_max;
elseif Fx_raw < Fx_min
    Fx_limited = Fx_min;
else
    Fx_limited = Fx_raw;
end

% =========================================================
% 9. 低速平滑权重
% =========================================================

vw = abs(Re_safe * omega_meas);

wv = (vw - v0) / (v1_safe - v0);

if wv > 1.0
    wv = 1.0;
elseif wv < 0.0
    wv = 0.0;
end

wv = wv * wv * (3.0 - 2.0 * wv);

Fx_weighted = wv * Fx_limited;

% =========================================================
% 10. 输出低通滤波
% =========================================================

if enable_lpf > 0.5
    alpha = exp(-Ts_safe / tau_safe);
    Fx_filt = alpha * Fx_filt + (1.0 - alpha) * Fx_weighted;
    Fx_est = Fx_filt;
else
    Fx_filt = Fx_weighted;
    Fx_est = Fx_weighted;
end

omega_hat_out = omega_hat;

end

== matlab function tractor_mu1109/驱动防滑模块/MATLAB Function3 ==
  data: vfl input; v output; vfr input; vrl input; vrr input; omega input; brk input; st input
function v = fcn(vfl,vfr,vrl,vrr,omega,brk,st)
d = 2.36;
brk_bank = 40;
st_bank = 10;

v = 0;
if abs(st) <= st_bank && brk < brk_bank
    v = min([vfl,vfr,vrl,vrr]);
elseif abs(st) <= st_bank && brk >= brk_bank
    v = max([vfl,vfr,vrl,vrr]);
elseif abs(st) > st_bank && brk >= brk_bank
    v = 0.5*max([vfl+vrl-d*omega,vfr+vrr+d*omega]);
elseif abs(st) > st_bank && brk < brk_bank
    v = 0.5*max([vfl+vrl-d*omega,vfr+vrr+d*omega]);
end

== matlab function tractor_mu1109/牵引效率计算/左前轮 ==
  data: Tw input; Fx_est output; omega_meas input; Fz input; Fx_raw output; Fx_limited output; omega_hat_out output; e_omega output; wv output
function [Fx_est, Fx_raw, Fx_limited, omega_hat_out, e_omega, wv] = ...
    FrontWheelFxObserver(Tw, omega_meas, Fz)

%#codegen
% 单轮纵向驱动力观测器
% 输入仅保留时变信号：
%   Tw         : 轮端驱动力矩 [N*m]
%   omega_meas : 实测车轮角速度 [rad/s]
%   Fz         : 单轮垂直载荷 [N]
%
% 输出：
%   Fx_est        : 最终纵向驱动力估计 [N]
%   Fx_raw        : 原始观测力估计 [N]
%   Fx_limited    : 限幅后力估计 [N]
%   omega_hat_out : 观测器内部估计轮速 [rad/s]
%   e_omega       : 轮速误差 [rad/s]
%   wv            : 低速平滑权重 [-]

% =========================================================
% 1. 固定参数区：根据具体车轮统一在这里调整
% =========================================================

Re = 0.834;              % 有效滚动半径 [m]
Jw = 110.64;            % 车轮等效转动惯量 [kg*m^2]
Ts = 0.001;             % 采样周期 [s]

mu = 0.7;               % 等效附着系数 [-]

l_omega = 50.0;         % 轮速误差反馈增益
fF = 3.0;               % 轮胎力观测带宽 [Hz]
gamma_F = Jw / Re * (2*pi*fF)^2;

enable_smc = 0;         % 是否启用滑模鲁棒项：1启用，0关闭
phi = 1.5;              % 滑模边界层厚度 [rad/s]
Func_ratio = 0.10;      % 未建模力比例，建议0.05~0.20
ks = Re / Jw * Func_ratio * mu * max(Fz, 0.0);

enable_lpf = 0;         % 是否启用输出低通：1启用，0关闭
tau_F = 0.08;           % 输出低通时间常数 [s]

v0 = 0.10;              % 低速权重起点 [m/s]
v1 = 0.80;              % 低速权重终点 [m/s]

eps_neg = 0.0;          % 允许负驱动力比例；严格驱动力估计取0
T_offset = 0.0;         % 轮端扭矩零偏 [N*m]
T_dead = 10.0;          % 扭矩死区 [N*m]

allow_brake_force = 0;  % 0：只估计驱动力；1：允许估计制动力

% =========================================================
% 2. 持久状态变量
% =========================================================

persistent omega_hat
persistent Fx_hat
persistent Fx_filt
persistent initialized

if isempty(initialized)
    omega_hat = 0.0;
    Fx_hat = 0.0;
    Fx_filt = 0.0;
    initialized = false;
end

if ~initialized
    omega_hat = omega_meas;
    Fx_hat = 0.0;
    Fx_filt = 0.0;
    initialized = true;
end

% =========================================================
% 3. 参数保护
% =========================================================

Jw_safe = max(Jw, 1e-6);
Re_safe = max(Re, 1e-6);
Ts_safe = max(Ts, 1e-6);
phi_safe = max(phi, 1e-6);
tau_safe = max(tau_F, Ts_safe);

Fz_safe = max(Fz, 0.0);
mu_safe = max(mu, 0.0);

if v1 <= v0
    v1_safe = v0 + 1e-3;
else
    v1_safe = v1;
end

% =========================================================
% 4. 扭矩零偏与死区处理
% =========================================================

Tw_corr = Tw - T_offset;

if abs(Tw_corr) < T_dead
    Tw_eff = 0.0;
else
    if Tw_corr > 0.0
        Tw_eff = Tw_corr - T_dead;
    else
        Tw_eff = Tw_corr + T_dead;
    end
end

if allow_brake_force < 0.5
    if Tw_eff < 0.0
        Tw_eff = 0.0;
    end
end

% =========================================================
% 5. 轮速误差
% =========================================================

e_omega = omega_meas - omega_hat;

% =========================================================
% 6. 滑模鲁棒项
% =========================================================

s = e_omega / phi_safe;

if s > 1.0
    sat_s = 1.0;
elseif s < -1.0
    sat_s = -1.0;
else
    sat_s = s;
end

if enable_smc > 0.5
    smc_term = ks * sat_s;
else
    smc_term = 0.0;
end

% =========================================================
% 7. 观测器状态更新
% =========================================================
%
% omega_hat_dot = Tw/Jw - Re/Jw*Fx_hat + l_omega*e_omega + ks*sat(e/phi)
% Fx_hat_dot    = -gamma_F*e_omega

omega_hat_dot = ...
    Tw_eff / Jw_safe ...
    - Re_safe / Jw_safe * Fx_hat ...
    + l_omega * e_omega ...
    + smc_term;

Fx_hat_dot = -gamma_F * e_omega;

omega_hat = omega_hat + Ts_safe * omega_hat_dot;
Fx_hat = Fx_hat + Ts_safe * Fx_hat_dot;

% =========================================================
% 8. 物理限幅与抗积分发散
% =========================================================

Fx_max = mu_safe * Fz_safe;

if allow_brake_force > 0.5
    Fx_min = -mu_safe * Fz_safe;
else
    Fx_min = -eps_neg * Fz_safe;
end

if Fx_hat > Fx_max
    Fx_hat = Fx_max;
elseif Fx_hat < Fx_min
    Fx_hat = Fx_min;
end

Fx_raw = Fx_hat;

if Fx_raw > Fx_max
    Fx_limited = Fx_max;
elseif Fx_raw < Fx_min
    Fx_limited = Fx_min;
else
    Fx_limited = Fx_raw;
end

% =========================================================
% 9. 低速平滑权重
% =========================================================

vw = abs(Re_safe * omega_meas);

wv = (vw - v0) / (v1_safe - v0);

if wv > 1.0
    wv = 1.0;
elseif wv < 0.0
    wv = 0.0;
end

wv = wv * wv * (3.0 - 2.0 * wv);

Fx_weighted = wv * Fx_limited;

% =========================================================
% 10. 输出低通滤波
% =========================================================

if enable_lpf > 0.5
    alpha = exp(-Ts_safe / tau_safe);
    Fx_filt = alpha * Fx_filt + (1.0 - alpha) * Fx_weighted;
    Fx_est = Fx_filt;
else
    Fx_filt = Fx_weighted;
    Fx_est = Fx_weighted;
end

omega_hat_out = omega_hat;

end

== matlab function tractor_mu1109/质心侧偏角滑模观测器估计/Subsystem/MATLAB Function ==
  data: vx input; d_vy_model output; delta_f input; vy_hat input; gamma_hat input; d_gamma_model output
function [d_vy_model, d_gamma_model] = fcn(vx, delta_f, vy_hat, gamma_hat)

% 声明我们将使用来自MATLAB基础工作区的参数
m = 18530;%质量
Iz = 67536;%绕Z轴的转动惯量
a = 2.043;%前轴距
b=1.362;%后轴距
% Cf = 1360400;%前侧偏刚度
% Cr = 1611200;%后侧偏刚度
 Cf = 304828*2;Cr = 417040*2; % 仿真用

% 防止vx为0导致计算错误
if abs(vx) < 0.1
    vx = 0.1;
end

% 二自由度模型方程
d_vy_model = (-(Cf + Cr) / (m * vx)) * vy_hat + ...
             ((b * Cr - a * Cf) / (m * vx) - vx) * gamma_hat + ...
             (Cf / m) * delta_f;

d_gamma_model = ((b * Cr - a * Cf) / (Iz * vx)) * vy_hat - ...
                ((a^2 * Cf + b^2 * Cr) / (Iz * vx)) * gamma_hat + ...
                (a * Cf / Iz) * delta_f;

== matlab function tractor_mu1109/质心侧偏角滑模观测器估计/Subsystem1/MATLAB Function ==
  data: vx input; d_vy_model output; delta_f input; vy_hat input; gamma_hat input; d_gamma_model output
function [d_vy_model, d_gamma_model] = fcn(vx, delta_f, vy_hat, gamma_hat)

% 声明我们将使用来自MATLAB基础工作区的参数
m = 18530;%质量
Iz = 67536;%绕Z轴的转动惯量
a = 2.043;%前轴距
b=1.362;%后轴距
Cf = 1360400;%前侧偏刚度
Cr = 1611200;%后侧偏刚度

% 防止vx为0导致计算错误
if abs(vx) < 0.1
    vx = 0.1;
end

% 二自由度模型方程
d_vy_model = (-(Cf + Cr) / (m * vx)) * vy_hat + ...
             ((b * Cr - a * Cf) / (m * vx) - vx) * gamma_hat + ...
             (Cf / m) * delta_f;

d_gamma_model = ((b * Cr - a * Cf) / (Iz * vx)) * vy_hat - ...
                ((a^2 * Cf + b^2 * Cr) / (Iz * vx)) * gamma_hat + ...
                (a * Cf / Iz) * delta_f;
